simulink model "ssc_hydromech_power_split_cvt_engine_signal_intf"  (R2025a)
settings: Solver=ode23t  StartTime=0.0  StopTime=70  RelTol=1e-3  AbsTol=1e-3
StartFcn:
  | tic
StopFcn:
  | Elapsed_Sim_Time = toc;
  | disp(['Elapsed Sim Time = ' num2str(Elapsed_Sim_Time)]);
undefined symbols (not defined in the file): DiscIntNeverNeededParam, HMPST, K, Lambda, tau, x0
libraries: fl_lib x30, nesl_utility x16, sm_wheel_loader_lib x9, simulink x7, simulink_extras x6, sdl_lib x3
(part 3 of 4)

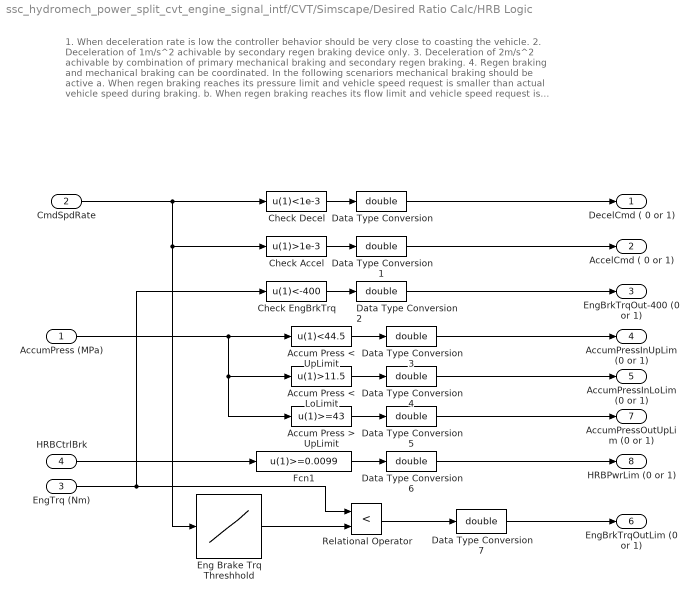
== system ssc_hydromech_power_split_cvt_engine_signal_intf/CVT/Simscape/Desired Ratio Calc/HRB Logic ==
  note: 1. When deceleration rate is low the controller behavior should be very close to coasting the vehicle.
      | 2. Deceleration of 1m/s^2 achivable by secondary regen braking device only.
      | 3. Deceleration of 2m/s^2 achivable by combination of primary mechanical braking and secondary regen braking.
      | 4. Regen braking and mechanical braking can be coordinated. In the following scenariors mechanical braking should be active
      | a. When regen braking reaches its pressure limit and vehicle speed request is smaller than actual vehicle speed during braking.
      | b. When regen braking reaches its flow limit and vehicle speed request is smaller than actual vehicle speed during braking.
      | 5. Energy in the accumulator will be released when accelerating and the accumulator pressure is above minimum working pressure.
      | Energy release rate should not cause engine over speeding.
      | 6. If engine over speed limit is reached disengage master clutch/shut down the engine.
  AccumPress (MPa) : Inport
  CmdSpdRate : Inport  Port=2
  EngTrq (Nm) : Inport  Port=3
  HRBCtrlBrk : Inport  Port=4
  Accum Press < LoLimit : Fcn  Expr=u(1)>11.5
  Accum Press < UpLimit : Fcn  Expr=u(1)<44.5
  Accum Press > UpLimit : Fcn  Expr=u(1)>=43
  Check Accel : Fcn  Expr=u(1)>1e-3
  Check Decel : Fcn  Expr=u(1)<1e-3
  Check EngBrkTrq : Fcn  Expr=u(1)<-400
  Data Type Conversion{,1..7} (8 alike) : DataTypeConversion  OutDataTypeStr=double  SaturateOnIntegerOverflow=off  RndMeth=Floor
  Eng Brake Trq Threshhold : Lookup_n-D  NumberOfTableDimensions=1  BreakpointsForDimension1=[-3 -2 -1 -0.5 0 1]  Table=[-450 -450 -225 -113 0 0]*0.6  InternalRulePriority=Speed  RndMeth=Simplest
  Fcn1 : Fcn  Expr=u(1)>=0.0099
  Relational Operator : RelationalOperator  Operator=<  OutDataTypeStr=boolean  ZeroCross=off  InputSameDT=off
  DecelCmd ( 0 or 1) : Outport
  AccelCmd ( 0 or 1) : Outport  Port=2
  EngBrkTrqOut-400 (0 or 1) : Outport  Port=3
  AccumPressInUpLim (0 or 1) : Outport  Port=4
  AccumPressInLoLim (0 or 1) : Outport  Port=5
  EngBrkTrqOutLim (0 or 1) : Outport  Port=6
  AccumPressOutUpLim (0 or 1) : Outport  Port=7
  HRBPwrLim (0 or 1) : Outport  Port=8
  wires:
  Data Type Conversion7/1 -> EngBrkTrqOutLim (0 or 1)/1
  Data Type Conversion6/1 -> HRBPwrLim (0 or 1)/1
  Data Type Conversion5/1 -> AccumPressOutUpLim (0 or 1)/1
  Data Type Conversion4/1 -> AccumPressInLoLim (0 or 1)/1
  Data Type Conversion3/1 -> AccumPressInUpLim (0 or 1)/1
  Data Type Conversion2/1 -> EngBrkTrqOut-400 (0 or 1)/1
  Data Type Conversion1/1 -> AccelCmd ( 0 or 1)/1
  Check EngBrkTrq/1 -> Data Type Conversion2/1
  Check Accel/1 -> Data Type Conversion1/1
  Accum Press < LoLimit/1 -> Data Type Conversion4/1
  Fcn1/1 -> Data Type Conversion6/1
  HRBCtrlBrk/1 -> Fcn1/1
  Accum Press > UpLimit/1 -> Data Type Conversion5/1
  Relational Operator/1 -> Data Type Conversion7/1
  Accum Press < UpLimit/1 -> Data Type Conversion3/1
  AccumPress (MPa)/1 -> Accum Press < UpLimit/1, Accum Press > UpLimit/1, Accum Press < LoLimit/1
  Eng Brake Trq Threshhold/1 -> Relational Operator/2
  CmdSpdRate/1 -> Check Accel/1, Eng Brake Trq Threshhold/1, Check Decel/1
  EngTrq (Nm)/1 -> Check EngBrkTrq/1, Relational Operator/1
  Data Type Conversion/1 -> DecelCmd ( 0 or 1)/1
  Check Decel/1 -> Data Type Conversion/1

== system ssc_hydromech_power_split_cvt_engine_signal_intf/CVT/Simscape/Desired Ratio Calc/MB Control ==
  Decel Error : Inport
  wTransOutCmd : Inport  Port=2
  Rset : Inport  Port=3
  AccumLimUp : Inport  Port=4
  HRBPowerLim : Inport  Port=5
  Add1 : Sum  Inputs=+++
  Compare To Constant : simulink/Logic and Bit Operations/Compare To Constant  relop=<=  const=0.02  OutDataTypeStr=boolean
  Data Type Conversion : DataTypeConversion  OutDataTypeStr=double  SaturateOnIntegerOverflow=off  RndMeth=Floor
  PI MB No HRB : Subsystem
  PI MB with MRB : Subsystem
  Product3 : Product  Inputs=3
  Product4 : Product
  Out1 : Outport
  wires:
  Decel Error/1 -> Product3/1, Product4/1
  Product3/1 -> PI MB No HRB/1(error)
  Rset/1 -> Product3/2, PI MB No HRB/2(Rset), PI MB with MRB/2(Rset)
  Compare To Constant/1 -> Data Type Conversion/1
  Data Type Conversion/1 -> Add1/1
  PI MB No HRB/1(ctrl) -> Add1/2
  Product4/1 -> PI MB with MRB/1(error)
  Add1/1 -> Out1/1
  PI MB with MRB/1(ctrl) -> Add1/3
  wTransOutCmd/1 -> Compare To Constant/1
  AccumLimUp/1 -> Product3/3
  HRBPowerLim/1 -> Product4/2

== system ssc_hydromech_power_split_cvt_engine_signal_intf/CVT/Simscape/Desired Ratio Calc/Subsystem ==
  u : Inport
  Constant1 : Constant
  Constant2 : Constant  Value=-1
  Constant3 : Constant  Value=0
  Gain : Gain  Gain=-1
  Switch : Switch  Criteria=u2 > Threshold  Threshold=0.001  SaturateOnIntegerOverflow=off  InputSameDT=off
  Switch1 : Switch  Criteria=u2 > Threshold  Threshold=0.001  SaturateOnIntegerOverflow=off  InputSameDT=off
  u_dir : Outport
  wires:
  Constant2/1 -> Switch1/1
  Constant3/1 -> Switch1/3
  Switch1/1 -> Switch/3
  Constant1/1 -> Switch/1
  u/1 -> Gain/1, Switch/2
  Switch/1 -> u_dir/1
  Gain/1 -> Switch1/2

== system ssc_hydromech_power_split_cvt_engine_signal_intf/CVT/Simscape/Port 1 Interface Engine/Interface ==
  across1 : Inport
  across2 : Inport  Port=2
  Continuous : Subsystem  VariantControl=Continuous
  Discrete : Subsystem  VariantControl=Discrete
  through2 : Outport
  through1 : Outport  Port=2

== system ssc_hydromech_power_split_cvt_engine_signal_intf/CVT/Simscape/Port 1 Interface Vehicle/Interface ==
  across1 : Inport
  across2 : Inport  Port=2
  Continuous : Subsystem  VariantControl=Continuous
  Discrete : Subsystem  VariantControl=Discrete
  through2 : Outport
  through1 : Outport  Port=2

== system ssc_hydromech_power_split_cvt_engine_signal_intf/CVT/Other/Desired Ratio Calc/HRB Control/PI HRB Brake ==
  error : Inport
  Rset : Inport  Port=2
  Gain : Gain  Gain=0.02*0.2
  Gain3 : Gain  Gain=0.002+0.0005
  Integrator : Integrator  ExternalReset=falling
  Sum : Sum  Inputs=++|
  ctrl : Outport
  wires:
  Rset/1 -> Integrator/2
  Integrator/1 -> Sum/1
  error/1 -> Gain3/1, Gain/1
  Sum/1 -> ctrl/1
  Gain3/1 -> Integrator/1
  Gain/1 -> Sum/2

== system ssc_hydromech_power_split_cvt_engine_signal_intf/CVT/Other/Desired Ratio Calc/HRB Control/PI HRB Regen ==
  error : Inport
  Rset : Inport  Port=2
  Gain : Gain  Gain=0.01*0.2
  Gain3 : Gain  Gain=0.001
  Integrator : Integrator  ExternalReset=falling
  Sum : Sum  Inputs=++|
  ctrl : Outport
  wires:
  Gain/1 -> Sum/2
  Gain3/1 -> Integrator/1
  Sum/1 -> ctrl/1
  error/1 -> Gain/1, Gain3/1
  Integrator/1 -> Sum/1
  Rset/1 -> Integrator/2

== system ssc_hydromech_power_split_cvt_engine_signal_intf/CVT/Other/Desired Ratio Calc/MB Control/PI MB No HRB ==
  error : Inport
  Rset : Inport  Port=2
  Gain : Gain  Gain=0.01
  Gain3 : Gain  Gain=0.002
  Integrator : Integrator  ExternalReset=falling
  Sum : Sum  Inputs=++|
  ctrl : Outport
  wires:
  Rset/1 -> Integrator/2
  Integrator/1 -> Sum/1
  error/1 -> Gain3/1, Gain/1
  Sum/1 -> ctrl/1
  Gain3/1 -> Integrator/1
  Gain/1 -> Sum/2

== system ssc_hydromech_power_split_cvt_engine_signal_intf/CVT/Other/Desired Ratio Calc/MB Control/PI MB with MRB ==
  error : Inport
  Rset : Inport  Port=2
  Gain : Gain  Gain=0.005
  Gain3 : Gain  Gain=0.002
  Integrator : Integrator  ExternalReset=falling
  Sum : Sum  Inputs=++|
  ctrl : Outport
  wires:
  Gain/1 -> Sum/2
  Gain3/1 -> Integrator/1
  Sum/1 -> ctrl/1
  error/1 -> Gain/1, Gain3/1
  Integrator/1 -> Sum/1
  Rset/1 -> Integrator/2

== system ssc_hydromech_power_split_cvt_engine_signal_intf/CVT/Other/Port 1 Interface Engine/Interface/Continuous ==
  across2 : Inport
  across1 : Inport  Port=2
  -1 : Gain  Gain=-1  SaturateOnIntegerOverflow=on  OutDataTypeStr=Inherit: Same as input  ParamDataTypeStr=Inherit: Same as input
  Integrator : Integrator  InitialCondition=x0
  K : Gain  Gain=K  SaturateOnIntegerOverflow=on  OutDataTypeStr=Inherit: Same as input  ParamDataTypeStr=Inherit: Same as input
  Lambda : Gain  Gain=Lambda  SaturateOnIntegerOverflow=on  OutDataTypeStr=Inherit: Same as input  ParamDataTypeStr=Inherit: Same as input
  Low-pass filter : TransferFcn  Numerator=1  Denominator=[tau 1]
  Prediction : Subsystem  Commented=through  mask(Prediction (discrete->continuous)){h2=h2}
      mask prompts: h2 "physmod:simscape:couplers:SimscapeNetworkCouplersLib:PortUDiscreteSampleTimes_MP"
      mask help: physmod:simscape:couplers:SimscapeNetworkCouplersLib:Predictiondiscretecontinuous_MD
      mask DialogControl h2 Prompt: Port u discrete sample time (s)
  Smoothing : Subsystem  Commented=through  mask(Smoothing (continuous->discrete)){tsSmoothing=tsSmoothing, smoothing0=-through0}
      mask prompts: tsSmoothing "physmod:simscape:couplers:SimscapeNetworkCouplersLib:SmoothingTimeConstants_MP"; smoothing0 "physmod:simscape:couplers:SimscapeNetworkCouplersLib:InitialOutput_MP"
      mask help: physmod:simscape:couplers:SimscapeNetworkCouplersLib:Smoothingcontinuousdiscrete_MD
      mask DialogControl tsSmoothing Prompt: Smoothing time constant (s)
      mask DialogControl smoothing0 Prompt: Initial output
  Sum : Sum  Inputs=+-  InputSameDT=on  SaturateOnIntegerOverflow=on  OutDataTypeStr=Inherit: Same as first input
  Sum2 : Sum  Inputs=|++
  through2 : Outport
  through1 : Outport  Port=2
  wires:
  K/1 -> Sum2/1
  Sum2/1 -> through1/1, -1/1
  across2/1 -> Prediction/1(u)
  Low-pass filter/1 -> Lambda/1
  Integrator/1 -> K/1
  Sum/1 -> Integrator/1, Low-pass filter/1
  across1/1 -> Sum/1
  Lambda/1 -> Sum2/2
  Prediction/1(y) -> Sum/2
  Smoothing/1(y) -> through2/1
  -1/1 -> Smoothing/1(u)

== system ssc_hydromech_power_split_cvt_engine_signal_intf/CVT/Other/Port 1 Interface Engine/Interface/Discrete ==
  across2 : Inport
  across1 : Inport  Port=2
  -1 : Gain  Gain=-1  SaturateOnIntegerOverflow=on  OutDataTypeStr=Inherit: Same as input  ParamDataTypeStr=Inherit: Same as input
  First-order lag : DiscreteTransferFcn  Numerator=h1  Denominator=[tau h1-tau]  SampleTime=h1
  Integrator : DiscreteIntegrator  InitialCondition=x0  SampleTime=h1  ICPrevOutput=DiscIntNeverNeededParam  ICPrevScaledInput=DiscIntNeverNeededParam
  K : Gain  Gain=K  SaturateOnIntegerOverflow=on  OutDataTypeStr=Inherit: Same as input  ParamDataTypeStr=Inherit: Same as input
  Lambda : Gain  Gain=Lambda  SaturateOnIntegerOverflow=on  OutDataTypeStr=Inherit: Same as input  ParamDataTypeStr=Inherit: Same as input
  Prediction : Subsystem  Commented=through  mask(Prediction (slow->fast)){h2=h2, h1=h1}
      mask prompts: h2 "physmod:simscape:couplers:SimscapeNetworkCouplersLib:PortUDiscreteSampleTimes_MP"; h1 "physmod:simscape:couplers:SimscapeNetworkCouplersLib:PortYDiscreteSampleTimes_MP"
      mask help: physmod:simscape:couplers:SimscapeNetworkCouplersLib:Predictionslowfast_MD
      mask DialogControl h2 Prompt: Port u discrete sample time (s)
      mask DialogControl h1 Prompt: Port y discrete sample time (s)
  Smoothing : Subsystem  Commented=through  mask(Smoothing (fast->slow)){nSmooth=nSmooth, h1=h1, smoothing0=-through0}
      mask prompts: nSmooth "physmod:simscape:couplers:SimscapeNetworkCouplersLib:NumberOfSamplesOverWhichToSmooth_MP"; h1 "physmod:simscape:couplers:SimscapeNetworkCouplersLib:PortUDiscreteSampleTimes_MP"; smoothing0 "physmod:simscape:couplers:SimscapeNetworkCouplersLib:InitialOutput_MP"
      mask help: physmod:simscape:couplers:SimscapeNetworkCouplersLib:Smoothingfastslow_MD
      mask DialogControl nSmooth Prompt: Number of samples over which to smooth
      mask DialogControl h1 Prompt: Port u discrete sample time (s)
      mask DialogControl smoothing0 Prompt: Initial output
  Sum : Sum  Inputs=+-  InputSameDT=on  SaturateOnIntegerOverflow=on  OutDataTypeStr=Inherit: Same as first input
  Sum1 : Sum  Inputs=|++
  through2 : Outport
  through1 : Outport  Port=2
  wires:
  First-order lag/1 -> Lambda/1
  Integrator/1 -> K/1
  K/1 -> Sum1/1
  across1/1 -> Sum/1
  Sum/1 -> Integrator/1, First-order lag/1
  across2/1 -> Prediction/1(u)
  Sum1/1 -> through1/1, -1/1
  Lambda/1 -> Sum1/2
  Prediction/1(y) -> Sum/2
  Smoothing/1(y) -> through2/1
  -1/1 -> Smoothing/1(u)

== system ssc_hydromech_power_split_cvt_engine_signal_intf/CVT/Other/Port 1 Interface Vehicle/Interface/Continuous ==
  across2 : Inport
  across1 : Inport  Port=2
  -1 : Gain  Gain=-1  SaturateOnIntegerOverflow=on  OutDataTypeStr=Inherit: Same as input  ParamDataTypeStr=Inherit: Same as input
  Integrator : Integrator  InitialCondition=x0
  K : Gain  Gain=K  SaturateOnIntegerOverflow=on  OutDataTypeStr=Inherit: Same as input  ParamDataTypeStr=Inherit: Same as input
  Lambda : Gain  Gain=Lambda  SaturateOnIntegerOverflow=on  OutDataTypeStr=Inherit: Same as input  ParamDataTypeStr=Inherit: Same as input
  Low-pass filter : TransferFcn  Numerator=1  Denominator=[tau 1]
  Prediction : Subsystem  Commented=through  mask(Prediction (discrete->continuous)){h2=h2}
      mask prompts: h2 "physmod:simscape:couplers:SimscapeNetworkCouplersLib:PortUDiscreteSampleTimes_MP"
      mask help: physmod:simscape:couplers:SimscapeNetworkCouplersLib:Predictiondiscretecontinuous_MD
      mask DialogControl h2 Prompt: Port u discrete sample time (s)
  Smoothing : Subsystem  Commented=through  mask(Smoothing (continuous->discrete)){tsSmoothing=tsSmoothing, smoothing0=-through0}
      mask prompts: tsSmoothing "physmod:simscape:couplers:SimscapeNetworkCouplersLib:SmoothingTimeConstants_MP"; smoothing0 "physmod:simscape:couplers:SimscapeNetworkCouplersLib:InitialOutput_MP"
      mask help: physmod:simscape:couplers:SimscapeNetworkCouplersLib:Smoothingcontinuousdiscrete_MD
      mask DialogControl tsSmoothing Prompt: Smoothing time constant (s)
      mask DialogControl smoothing0 Prompt: Initial output
  Sum : Sum  Inputs=+-  InputSameDT=on  SaturateOnIntegerOverflow=on  OutDataTypeStr=Inherit: Same as first input
  Sum2 : Sum  Inputs=|++
  through2 : Outport
  through1 : Outport  Port=2
  wires:
  K/1 -> Sum2/1
  Sum2/1 -> through1/1, -1/1
  across2/1 -> Prediction/1(u)
  Low-pass filter/1 -> Lambda/1
  Integrator/1 -> K/1
  Sum/1 -> Integrator/1, Low-pass filter/1
  across1/1 -> Sum/1
  Lambda/1 -> Sum2/2
  Prediction/1(y) -> Sum/2
  Smoothing/1(y) -> through2/1
  -1/1 -> Smoothing/1(u)

== system ssc_hydromech_power_split_cvt_engine_signal_intf/CVT/Other/Port 1 Interface Vehicle/Interface/Discrete ==
  across2 : Inport
  across1 : Inport  Port=2
  -1 : Gain  Gain=-1  SaturateOnIntegerOverflow=on  OutDataTypeStr=Inherit: Same as input  ParamDataTypeStr=Inherit: Same as input
  First-order lag : DiscreteTransferFcn  Numerator=h1  Denominator=[tau h1-tau]  SampleTime=h1
  Integrator : DiscreteIntegrator  InitialCondition=x0  SampleTime=h1  ICPrevOutput=DiscIntNeverNeededParam  ICPrevScaledInput=DiscIntNeverNeededParam
  K : Gain  Gain=K  SaturateOnIntegerOverflow=on  OutDataTypeStr=Inherit: Same as input  ParamDataTypeStr=Inherit: Same as input
  Lambda : Gain  Gain=Lambda  SaturateOnIntegerOverflow=on  OutDataTypeStr=Inherit: Same as input  ParamDataTypeStr=Inherit: Same as input
  Prediction : Subsystem  Commented=through  mask(Prediction (slow->fast)){h2=h2, h1=h1}
      mask prompts: h2 "physmod:simscape:couplers:SimscapeNetworkCouplersLib:PortUDiscreteSampleTimes_MP"; h1 "physmod:simscape:couplers:SimscapeNetworkCouplersLib:PortYDiscreteSampleTimes_MP"
      mask help: physmod:simscape:couplers:SimscapeNetworkCouplersLib:Predictionslowfast_MD
      mask DialogControl h2 Prompt: Port u discrete sample time (s)
      mask DialogControl h1 Prompt: Port y discrete sample time (s)
  Smoothing : Subsystem  Commented=through  mask(Smoothing (fast->slow)){nSmooth=nSmooth, h1=h1, smoothing0=-through0}
      mask prompts: nSmooth "physmod:simscape:couplers:SimscapeNetworkCouplersLib:NumberOfSamplesOverWhichToSmooth_MP"; h1 "physmod:simscape:couplers:SimscapeNetworkCouplersLib:PortUDiscreteSampleTimes_MP"; smoothing0 "physmod:simscape:couplers:SimscapeNetworkCouplersLib:InitialOutput_MP"
      mask help: physmod:simscape:couplers:SimscapeNetworkCouplersLib:Smoothingfastslow_MD
      mask DialogControl nSmooth Prompt: Number of samples over which to smooth
      mask DialogControl h1 Prompt: Port u discrete sample time (s)
      mask DialogControl smoothing0 Prompt: Initial output
  Sum : Sum  Inputs=+-  InputSameDT=on  SaturateOnIntegerOverflow=on  OutDataTypeStr=Inherit: Same as first input
  Sum1 : Sum  Inputs=|++
  through2 : Outport
  through1 : Outport  Port=2
  wires:
  First-order lag/1 -> Lambda/1
  Integrator/1 -> K/1
  K/1 -> Sum1/1
  across1/1 -> Sum/1
  Sum/1 -> Integrator/1, First-order lag/1
  across2/1 -> Prediction/1(u)
  Sum1/1 -> through1/1, -1/1
  Lambda/1 -> Sum1/2
  Prediction/1(y) -> Sum/2
  Smoothing/1(y) -> through2/1
  -1/1 -> Smoothing/1(u)

== system ssc_hydromech_power_split_cvt_engine_signal_intf/CVT/Simscape/Desired Ratio Calc/HRB Control/PI HRB Brake ==
  error : Inport
  Rset : Inport  Port=2
  Gain : Gain  Gain=0.02*0.2
  Gain3 : Gain  Gain=0.002+0.0005
  Integrator : Integrator  ExternalReset=falling
  Sum : Sum  Inputs=++|
  ctrl : Outport
  wires:
  Gain/1 -> Sum/2
  Gain3/1 -> Integrator/1
  Sum/1 -> ctrl/1
  error/1 -> Gain/1, Gain3/1
  Integrator/1 -> Sum/1
  Rset/1 -> Integrator/2

== system ssc_hydromech_power_split_cvt_engine_signal_intf/CVT/Simscape/Desired Ratio Calc/HRB Control/PI HRB Regen ==
  error : Inport
  Rset : Inport  Port=2
  Gain : Gain  Gain=0.01*0.2
  Gain3 : Gain  Gain=0.001
  Integrator : Integrator  ExternalReset=falling
  Sum : Sum  Inputs=++|
  ctrl : Outport
  wires:
  Rset/1 -> Integrator/2
  Integrator/1 -> Sum/1
  error/1 -> Gain3/1, Gain/1
  Sum/1 -> ctrl/1
  Gain3/1 -> Integrator/1
  Gain/1 -> Sum/2

== system ssc_hydromech_power_split_cvt_engine_signal_intf/CVT/Simscape/Desired Ratio Calc/MB Control/PI MB No HRB ==
  error : Inport
  Rset : Inport  Port=2
  Gain : Gain  Gain=0.01
  Gain3 : Gain  Gain=0.002
  Integrator : Integrator  ExternalReset=falling
  Sum : Sum  Inputs=++|
  ctrl : Outport
  wires:
  Gain/1 -> Sum/2
  Gain3/1 -> Integrator/1
  Sum/1 -> ctrl/1
  error/1 -> Gain/1, Gain3/1
  Integrator/1 -> Sum/1
  Rset/1 -> Integrator/2

== system ssc_hydromech_power_split_cvt_engine_signal_intf/CVT/Simscape/Desired Ratio Calc/MB Control/PI MB with MRB ==
  error : Inport
  Rset : Inport  Port=2
  Gain : Gain  Gain=0.005
  Gain3 : Gain  Gain=0.002
  Integrator : Integrator  ExternalReset=falling
  Sum : Sum  Inputs=++|
  ctrl : Outport
  wires:
  Rset/1 -> Integrator/2
  Integrator/1 -> Sum/1
  error/1 -> Gain3/1, Gain/1
  Sum/1 -> ctrl/1
  Gain3/1 -> Integrator/1
  Gain/1 -> Sum/2

== system ssc_hydromech_power_split_cvt_engine_signal_intf/CVT/Simscape/Port 1 Interface Engine/Interface/Continuous ==
  across2 : Inport
  across1 : Inport  Port=2
  -1 : Gain  Gain=-1  SaturateOnIntegerOverflow=on  OutDataTypeStr=Inherit: Same as input  ParamDataTypeStr=Inherit: Same as input
  Integrator : Integrator  InitialCondition=x0
  K : Gain  Gain=K  SaturateOnIntegerOverflow=on  OutDataTypeStr=Inherit: Same as input  ParamDataTypeStr=Inherit: Same as input
  Lambda : Gain  Gain=Lambda  SaturateOnIntegerOverflow=on  OutDataTypeStr=Inherit: Same as input  ParamDataTypeStr=Inherit: Same as input
  Low-pass filter : TransferFcn  Numerator=1  Denominator=[tau 1]
  Prediction : Subsystem  Commented=through  mask(Prediction (discrete->continuous)){h2=h2}
      mask prompts: h2 "physmod:simscape:couplers:SimscapeNetworkCouplersLib:PortUDiscreteSampleTimes_MP"
      mask help: physmod:simscape:couplers:SimscapeNetworkCouplersLib:Predictiondiscretecontinuous_MD
      mask DialogControl h2 Prompt: Port u discrete sample time (s)
  Smoothing : Subsystem  Commented=through  mask(Smoothing (continuous->discrete)){tsSmoothing=tsSmoothing, smoothing0=-through0}
      mask prompts: tsSmoothing "physmod:simscape:couplers:SimscapeNetworkCouplersLib:SmoothingTimeConstants_MP"; smoothing0 "physmod:simscape:couplers:SimscapeNetworkCouplersLib:InitialOutput_MP"
      mask help: physmod:simscape:couplers:SimscapeNetworkCouplersLib:Smoothingcontinuousdiscrete_MD
      mask DialogControl tsSmoothing Prompt: Smoothing time constant (s)
      mask DialogControl smoothing0 Prompt: Initial output
  Sum : Sum  Inputs=+-  InputSameDT=on  SaturateOnIntegerOverflow=on  OutDataTypeStr=Inherit: Same as first input
  Sum2 : Sum  Inputs=|++
  through2 : Outport
  through1 : Outport  Port=2
  wires:
  -1/1 -> Smoothing/1(u)
  Smoothing/1(y) -> through2/1
  Prediction/1(y) -> Sum/2
  Lambda/1 -> Sum2/2
  across1/1 -> Sum/1
  Sum/1 -> Low-pass filter/1, Integrator/1
  Integrator/1 -> K/1
  Low-pass filter/1 -> Lambda/1
  across2/1 -> Prediction/1(u)
  Sum2/1 -> -1/1, through1/1
  K/1 -> Sum2/1

== system ssc_hydromech_power_split_cvt_engine_signal_intf/CVT/Simscape/Port 1 Interface Engine/Interface/Discrete ==
  across2 : Inport
  across1 : Inport  Port=2
  -1 : Gain  Gain=-1  SaturateOnIntegerOverflow=on  OutDataTypeStr=Inherit: Same as input  ParamDataTypeStr=Inherit: Same as input
  First-order lag : DiscreteTransferFcn  Numerator=h1  Denominator=[tau h1-tau]  SampleTime=h1
  Integrator : DiscreteIntegrator  InitialCondition=x0  SampleTime=h1  ICPrevOutput=DiscIntNeverNeededParam  ICPrevScaledInput=DiscIntNeverNeededParam
  K : Gain  Gain=K  SaturateOnIntegerOverflow=on  OutDataTypeStr=Inherit: Same as input  ParamDataTypeStr=Inherit: Same as input
  Lambda : Gain  Gain=Lambda  SaturateOnIntegerOverflow=on  OutDataTypeStr=Inherit: Same as input  ParamDataTypeStr=Inherit: Same as input
  Prediction : Subsystem  Commented=through  mask(Prediction (slow->fast)){h2=h2, h1=h1}
      mask prompts: h2 "physmod:simscape:couplers:SimscapeNetworkCouplersLib:PortUDiscreteSampleTimes_MP"; h1 "physmod:simscape:couplers:SimscapeNetworkCouplersLib:PortYDiscreteSampleTimes_MP"
      mask help: physmod:simscape:couplers:SimscapeNetworkCouplersLib:Predictionslowfast_MD
      mask DialogControl h2 Prompt: Port u discrete sample time (s)
      mask DialogControl h1 Prompt: Port y discrete sample time (s)
  Smoothing : Subsystem  Commented=through  mask(Smoothing (fast->slow)){nSmooth=nSmooth, h1=h1, smoothing0=-through0}
      mask prompts: nSmooth "physmod:simscape:couplers:SimscapeNetworkCouplersLib:NumberOfSamplesOverWhichToSmooth_MP"; h1 "physmod:simscape:couplers:SimscapeNetworkCouplersLib:PortUDiscreteSampleTimes_MP"; smoothing0 "physmod:simscape:couplers:SimscapeNetworkCouplersLib:InitialOutput_MP"
      mask help: physmod:simscape:couplers:SimscapeNetworkCouplersLib:Smoothingfastslow_MD
      mask DialogControl nSmooth Prompt: Number of samples over which to smooth
      mask DialogControl h1 Prompt: Port u discrete sample time (s)
      mask DialogControl smoothing0 Prompt: Initial output
  Sum : Sum  Inputs=+-  InputSameDT=on  SaturateOnIntegerOverflow=on  OutDataTypeStr=Inherit: Same as first input
  Sum1 : Sum  Inputs=|++
  through2 : Outport
  through1 : Outport  Port=2
  wires:
  -1/1 -> Smoothing/1(u)
  Smoothing/1(y) -> through2/1
  Prediction/1(y) -> Sum/2
  Lambda/1 -> Sum1/2
  Sum1/1 -> -1/1, through1/1
  across2/1 -> Prediction/1(u)
  Sum/1 -> First-order lag/1, Integrator/1
  across1/1 -> Sum/1
  K/1 -> Sum1/1
  Integrator/1 -> K/1
  First-order lag/1 -> Lambda/1

== system ssc_hydromech_power_split_cvt_engine_signal_intf/CVT/Simscape/Port 1 Interface Vehicle/Interface/Continuous ==
  across2 : Inport
  across1 : Inport  Port=2
  -1 : Gain  Gain=-1  SaturateOnIntegerOverflow=on  OutDataTypeStr=Inherit: Same as input  ParamDataTypeStr=Inherit: Same as input
  Integrator : Integrator  InitialCondition=x0
  K : Gain  Gain=K  SaturateOnIntegerOverflow=on  OutDataTypeStr=Inherit: Same as input  ParamDataTypeStr=Inherit: Same as input
  Lambda : Gain  Gain=Lambda  SaturateOnIntegerOverflow=on  OutDataTypeStr=Inherit: Same as input  ParamDataTypeStr=Inherit: Same as input
  Low-pass filter : TransferFcn  Numerator=1  Denominator=[tau 1]
  Prediction : Subsystem  Commented=through  mask(Prediction (discrete->continuous)){h2=h2}
      mask prompts: h2 "physmod:simscape:couplers:SimscapeNetworkCouplersLib:PortUDiscreteSampleTimes_MP"
      mask help: physmod:simscape:couplers:SimscapeNetworkCouplersLib:Predictiondiscretecontinuous_MD
      mask DialogControl h2 Prompt: Port u discrete sample time (s)
  Smoothing : Subsystem  Commented=through  mask(Smoothing (continuous->discrete)){tsSmoothing=tsSmoothing, smoothing0=-through0}
      mask prompts: tsSmoothing "physmod:simscape:couplers:SimscapeNetworkCouplersLib:SmoothingTimeConstants_MP"; smoothing0 "physmod:simscape:couplers:SimscapeNetworkCouplersLib:InitialOutput_MP"
      mask help: physmod:simscape:couplers:SimscapeNetworkCouplersLib:Smoothingcontinuousdiscrete_MD
      mask DialogControl tsSmoothing Prompt: Smoothing time constant (s)
      mask DialogControl smoothing0 Prompt: Initial output
  Sum : Sum  Inputs=+-  InputSameDT=on  SaturateOnIntegerOverflow=on  OutDataTypeStr=Inherit: Same as first input
  Sum2 : Sum  Inputs=|++
  through2 : Outport
  through1 : Outport  Port=2
  wires:
  -1/1 -> Smoothing/1(u)
  Smoothing/1(y) -> through2/1
  Prediction/1(y) -> Sum/2
  Lambda/1 -> Sum2/2
  across1/1 -> Sum/1
  Sum/1 -> Low-pass filter/1, Integrator/1
  Integrator/1 -> K/1
  Low-pass filter/1 -> Lambda/1
  across2/1 -> Prediction/1(u)
  Sum2/1 -> -1/1, through1/1
  K/1 -> Sum2/1

== system ssc_hydromech_power_split_cvt_engine_signal_intf/CVT/Simscape/Port 1 Interface Vehicle/Interface/Discrete ==
  across2 : Inport
  across1 : Inport  Port=2
  -1 : Gain  Gain=-1  SaturateOnIntegerOverflow=on  OutDataTypeStr=Inherit: Same as input  ParamDataTypeStr=Inherit: Same as input
  First-order lag : DiscreteTransferFcn  Numerator=h1  Denominator=[tau h1-tau]  SampleTime=h1
  Integrator : DiscreteIntegrator  InitialCondition=x0  SampleTime=h1  ICPrevOutput=DiscIntNeverNeededParam  ICPrevScaledInput=DiscIntNeverNeededParam
  K : Gain  Gain=K  SaturateOnIntegerOverflow=on  OutDataTypeStr=Inherit: Same as input  ParamDataTypeStr=Inherit: Same as input
  Lambda : Gain  Gain=Lambda  SaturateOnIntegerOverflow=on  OutDataTypeStr=Inherit: Same as input  ParamDataTypeStr=Inherit: Same as input
  Prediction : Subsystem  Commented=through  mask(Prediction (slow->fast)){h2=h2, h1=h1}
      mask prompts: h2 "physmod:simscape:couplers:SimscapeNetworkCouplersLib:PortUDiscreteSampleTimes_MP"; h1 "physmod:simscape:couplers:SimscapeNetworkCouplersLib:PortYDiscreteSampleTimes_MP"
      mask help: physmod:simscape:couplers:SimscapeNetworkCouplersLib:Predictionslowfast_MD
      mask DialogControl h2 Prompt: Port u discrete sample time (s)
      mask DialogControl h1 Prompt: Port y discrete sample time (s)
  Smoothing : Subsystem  Commented=through  mask(Smoothing (fast->slow)){nSmooth=nSmooth, h1=h1, smoothing0=-through0}
      mask prompts: nSmooth "physmod:simscape:couplers:SimscapeNetworkCouplersLib:NumberOfSamplesOverWhichToSmooth_MP"; h1 "physmod:simscape:couplers:SimscapeNetworkCouplersLib:PortUDiscreteSampleTimes_MP"; smoothing0 "physmod:simscape:couplers:SimscapeNetworkCouplersLib:InitialOutput_MP"
      mask help: physmod:simscape:couplers:SimscapeNetworkCouplersLib:Smoothingfastslow_MD
      mask DialogControl nSmooth Prompt: Number of samples over which to smooth
      mask DialogControl h1 Prompt: Port u discrete sample time (s)
      mask DialogControl smoothing0 Prompt: Initial output
  Sum : Sum  Inputs=+-  InputSameDT=on  SaturateOnIntegerOverflow=on  OutDataTypeStr=Inherit: Same as first input
  Sum1 : Sum  Inputs=|++
  through2 : Outport
  through1 : Outport  Port=2
  wires:
  -1/1 -> Smoothing/1(u)
  Smoothing/1(y) -> through2/1
  Prediction/1(y) -> Sum/2
  Lambda/1 -> Sum1/2
  Sum1/1 -> -1/1, through1/1
  across2/1 -> Prediction/1(u)
  Sum/1 -> First-order lag/1, Integrator/1
  across1/1 -> Sum/1
  K/1 -> Sum1/1
  Integrator/1 -> K/1
  First-order lag/1 -> Lambda/1

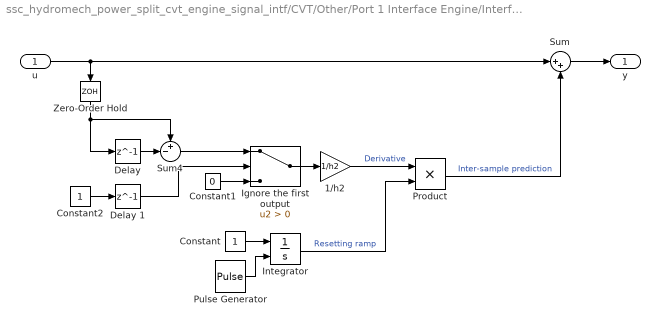
== system ssc_hydromech_power_split_cvt_engine_signal_intf/CVT/Other/Port 1 Interface Engine/Interface/Continuous/Prediction ==
  u : Inport
  1/h2 : Gain  Gain=1/h2
  Constant : Constant  SampleTime=h2
  Constant1 : Constant  Value=0  SampleTime=h2
  Constant2 : Constant  SampleTime=h2
  "Delay " : Delay  DelayLength=1  SampleTime=h2
  Delay 1 : Delay  DelayLength=1  SampleTime=h2
  Ignore the first output : Switch  Criteria=u2 > Threshold  SaturateOnIntegerOverflow=off  InputSameDT=off
  Integrator : Integrator  ExternalReset=either  LimitOutput=on  UpperSaturationLimit=1  LowerSaturationLimit=0
  Product : Product
  Pulse Generator : DiscretePulseGenerator  SampleTime=h2
  Sum : Sum  Inputs=|++
  Sum4 : Sum  Inputs=+-|
  Zero-Order Hold : ZeroOrderHold  SampleTime=h2
  y : Outport
  wires:
  Product/1 -> Sum/2  "Inter-sample prediction"
  Zero-Order Hold/1 -> Sum4/1, "Delay "/1
  u/1 -> Sum/1, Zero-Order Hold/1
  "Delay "/1 -> Sum4/2
  1/h2/1 -> Product/1  "Derivative"
  Sum/1 -> y/1
  Integrator/1 -> Product/2  "Resetting ramp"
  Constant/1 -> Integrator/1
  Pulse Generator/1 -> Integrator/2
  Ignore the first output/1 -> 1/h2/1
  Sum4/1 -> Ignore the first output/1
  Constant1/1 -> Ignore the first output/3
  Delay 1/1 -> Ignore the first output/2
  Constant2/1 -> Delay 1/1

== system ssc_hydromech_power_split_cvt_engine_signal_intf/CVT/Other/Port 1 Interface Engine/Interface/Continuous/Smoothing ==
  u : Inport
  Gain : Gain  Gain=1/tsSmoothing
  Integrator : Integrator  InitialCondition=smoothing0
  Sum : Sum  Inputs=|+-
  y : Outport
  wires:
  u/1 -> Sum/1
  Integrator/1 -> Sum/2, y/1
  Gain/1 -> Integrator/1
  Sum/1 -> Gain/1

== system ssc_hydromech_power_split_cvt_engine_signal_intf/CVT/Other/Port 1 Interface Engine/Interface/Discrete/Prediction ==
  u : Inport
  Abs : Abs  SaturateOnIntegerOverflow=off
  Constant : Constant  Value=0  SampleTime=h1
  Constant2 : Constant  Value=h1  SampleTime=h1
  "Delay " : Delay  DelayLength=1  SampleTime=h1
  Product : Product
  Resettable Delay : Delay  DelayLength=1  InitialConditionSource=Input port  ExternalReset=Rising  SampleTime=h1
      settings: InputPortMap=u0,r5,p4
  Sum : Sum  Inputs=|++
  Sum1 : Sum  Inputs=|++
  Sum2 : Sum  Inputs=+
  Sum4 : Sum  Inputs=+-|
  Update derivative estimate : Subsystem  TreatAsAtomicUnit=on
  y : Outport
  wires:
  Abs/1 -> Sum2/1
  Sum2/1 -> Resettable Delay/2, Update derivative estimate/Trigger  "Trigger when input changes"
  Sum1/1 -> Resettable Delay/1
  Sum/1 -> y/1
  "Delay "/1 -> Sum4/2
  Product/1 -> Sum/2
  Update derivative estimate/1(Out1) -> Product/1
  u/1 -> Update derivative estimate/1(u), "Delay "/1, Sum/1, Sum4/1
  Sum4/1 -> Abs/1
  Resettable Delay/1 -> Product/2, Sum1/2
  Constant2/1 -> Sum1/1
  Constant/1 -> Resettable Delay/3

== system ssc_hydromech_power_split_cvt_engine_signal_intf/CVT/Other/Port 1 Interface Engine/Interface/Discrete/Smoothing ==
  u : Inport
  Gain : Gain  Gain=1/nSmooth
  Sum of Elements : Sum  Inputs=+
  Tapped Delay : simulink/Discrete/Tapped Delay  vinit=smoothing0  samptime=h1  NumDelays=nSmooth  DelayOrder=Oldest  includeCurrent=off
  y : Outport
  wires:
  Gain/1 -> y/1
  Sum of Elements/1 -> Gain/1
  Tapped Delay/1 -> Sum of Elements/1
  u/1 -> Tapped Delay/1

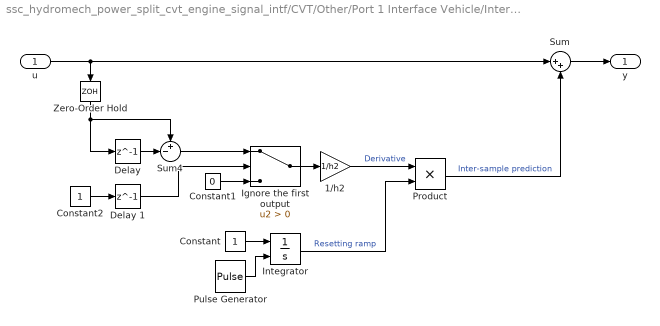
== system ssc_hydromech_power_split_cvt_engine_signal_intf/CVT/Other/Port 1 Interface Vehicle/Interface/Continuous/Prediction ==
  u : Inport
  1/h2 : Gain  Gain=1/h2
  Constant : Constant  SampleTime=h2
  Constant1 : Constant  Value=0  SampleTime=h2
  Constant2 : Constant  SampleTime=h2
  "Delay " : Delay  DelayLength=1  SampleTime=h2
  Delay 1 : Delay  DelayLength=1  SampleTime=h2
  Ignore the first output : Switch  Criteria=u2 > Threshold  SaturateOnIntegerOverflow=off  InputSameDT=off
  Integrator : Integrator  ExternalReset=either  LimitOutput=on  UpperSaturationLimit=1  LowerSaturationLimit=0
  Product : Product
  Pulse Generator : DiscretePulseGenerator  SampleTime=h2
  Sum : Sum  Inputs=|++
  Sum4 : Sum  Inputs=+-|
  Zero-Order Hold : ZeroOrderHold  SampleTime=h2
  y : Outport
  wires:
  Product/1 -> Sum/2  "Inter-sample prediction"
  Zero-Order Hold/1 -> Sum4/1, "Delay "/1
  u/1 -> Sum/1, Zero-Order Hold/1
  "Delay "/1 -> Sum4/2
  1/h2/1 -> Product/1  "Derivative"
  Sum/1 -> y/1
  Integrator/1 -> Product/2  "Resetting ramp"
  Constant/1 -> Integrator/1
  Pulse Generator/1 -> Integrator/2
  Ignore the first output/1 -> 1/h2/1
  Sum4/1 -> Ignore the first output/1
  Constant1/1 -> Ignore the first output/3
  Delay 1/1 -> Ignore the first output/2
  Constant2/1 -> Delay 1/1

== system ssc_hydromech_power_split_cvt_engine_signal_intf/CVT/Other/Port 1 Interface Vehicle/Interface/Continuous/Smoothing ==
  u : Inport
  Gain : Gain  Gain=1/tsSmoothing
  Integrator : Integrator  InitialCondition=smoothing0
  Sum : Sum  Inputs=|+-
  y : Outport
  wires:
  u/1 -> Sum/1
  Integrator/1 -> Sum/2, y/1
  Gain/1 -> Integrator/1
  Sum/1 -> Gain/1

== system ssc_hydromech_power_split_cvt_engine_signal_intf/CVT/Other/Port 1 Interface Vehicle/Interface/Discrete/Prediction ==
  u : Inport
  Abs : Abs  SaturateOnIntegerOverflow=off
  Constant : Constant  Value=0  SampleTime=h1
  Constant2 : Constant  Value=h1  SampleTime=h1
  "Delay " : Delay  DelayLength=1  SampleTime=h1
  Product : Product
  Resettable Delay : Delay  DelayLength=1  InitialConditionSource=Input port  ExternalReset=Rising  SampleTime=h1
      settings: InputPortMap=u0,r5,p4
  Sum : Sum  Inputs=|++
  Sum1 : Sum  Inputs=|++
  Sum2 : Sum  Inputs=+
  Sum4 : Sum  Inputs=+-|
  Update derivative estimate : Subsystem  TreatAsAtomicUnit=on
  y : Outport
  wires:
  Abs/1 -> Sum2/1
  Sum2/1 -> Resettable Delay/2, Update derivative estimate/Trigger  "Trigger when input changes"
  Sum1/1 -> Resettable Delay/1
  Sum/1 -> y/1
  "Delay "/1 -> Sum4/2
  Product/1 -> Sum/2
  Update derivative estimate/1(Out1) -> Product/1
  u/1 -> Update derivative estimate/1(u), "Delay "/1, Sum/1, Sum4/1
  Sum4/1 -> Abs/1
  Resettable Delay/1 -> Product/2, Sum1/2
  Constant2/1 -> Sum1/1
  Constant/1 -> Resettable Delay/3

== system ssc_hydromech_power_split_cvt_engine_signal_intf/CVT/Other/Port 1 Interface Vehicle/Interface/Discrete/Smoothing ==
  u : Inport
  Gain : Gain  Gain=1/nSmooth
  Sum of Elements : Sum  Inputs=+
  Tapped Delay : simulink/Discrete/Tapped Delay  vinit=smoothing0  samptime=h1  NumDelays=nSmooth  DelayOrder=Oldest  includeCurrent=off
  y : Outport
  wires:
  Gain/1 -> y/1
  Sum of Elements/1 -> Gain/1
  Tapped Delay/1 -> Sum of Elements/1
  u/1 -> Tapped Delay/1

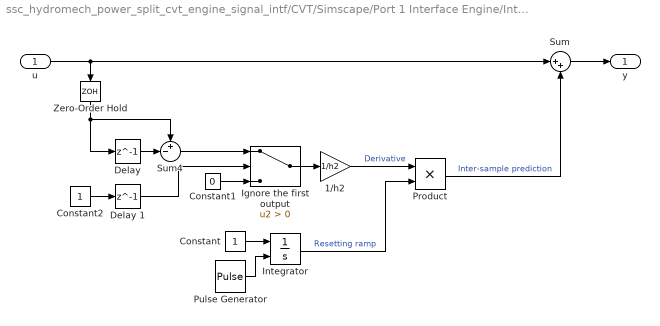
== system ssc_hydromech_power_split_cvt_engine_signal_intf/CVT/Simscape/Port 1 Interface Engine/Interface/Continuous/Prediction ==
  u : Inport
  1/h2 : Gain  Gain=1/h2
  Constant : Constant  SampleTime=h2
  Constant1 : Constant  Value=0  SampleTime=h2
  Constant2 : Constant  SampleTime=h2
  "Delay " : Delay  DelayLength=1  SampleTime=h2
  Delay 1 : Delay  DelayLength=1  SampleTime=h2
  Ignore the first output : Switch  Criteria=u2 > Threshold  SaturateOnIntegerOverflow=off  InputSameDT=off
  Integrator : Integrator  ExternalReset=either  LimitOutput=on  UpperSaturationLimit=1  LowerSaturationLimit=0
  Product : Product
  Pulse Generator : DiscretePulseGenerator  SampleTime=h2
  Sum : Sum  Inputs=|++
  Sum4 : Sum  Inputs=+-|
  Zero-Order Hold : ZeroOrderHold  SampleTime=h2
  y : Outport
  wires:
  Constant2/1 -> Delay 1/1
  Delay 1/1 -> Ignore the first output/2
  Constant1/1 -> Ignore the first output/3
  Sum4/1 -> Ignore the first output/1
  Ignore the first output/1 -> 1/h2/1
  Pulse Generator/1 -> Integrator/2
  Constant/1 -> Integrator/1
  Integrator/1 -> Product/2  "Resetting ramp"
  Sum/1 -> y/1
  1/h2/1 -> Product/1  "Derivative"
  "Delay "/1 -> Sum4/2
  u/1 -> Zero-Order Hold/1, Sum/1
  Zero-Order Hold/1 -> "Delay "/1, Sum4/1
  Product/1 -> Sum/2  "Inter-sample prediction"

== system ssc_hydromech_power_split_cvt_engine_signal_intf/CVT/Simscape/Port 1 Interface Engine/Interface/Continuous/Smoothing ==
  u : Inport
  Gain : Gain  Gain=1/tsSmoothing
  Integrator : Integrator  InitialCondition=smoothing0
  Sum : Sum  Inputs=|+-
  y : Outport
  wires:
  Sum/1 -> Gain/1
  Gain/1 -> Integrator/1
  Integrator/1 -> y/1, Sum/2
  u/1 -> Sum/1

== system ssc_hydromech_power_split_cvt_engine_signal_intf/CVT/Simscape/Port 1 Interface Engine/Interface/Discrete/Prediction ==
  u : Inport
  Abs : Abs  SaturateOnIntegerOverflow=off
  Constant : Constant  Value=0  SampleTime=h1
  Constant2 : Constant  Value=h1  SampleTime=h1
  "Delay " : Delay  DelayLength=1  SampleTime=h1
  Product : Product
  Resettable Delay : Delay  DelayLength=1  InitialConditionSource=Input port  ExternalReset=Rising  SampleTime=h1
      settings: InputPortMap=u0,r5,p4
  Sum : Sum  Inputs=|++
  Sum1 : Sum  Inputs=|++
  Sum2 : Sum  Inputs=+
  Sum4 : Sum  Inputs=+-|
  Update derivative estimate : Subsystem  TreatAsAtomicUnit=on
  y : Outport
  wires:
  Constant/1 -> Resettable Delay/3
  Constant2/1 -> Sum1/1
  Resettable Delay/1 -> Sum1/2, Product/2
  Sum4/1 -> Abs/1
  u/1 -> Sum4/1, Sum/1, "Delay "/1, Update derivative estimate/1(u)
  Update derivative estimate/1(Out1) -> Product/1
  Product/1 -> Sum/2
  "Delay "/1 -> Sum4/2
  Sum/1 -> y/1
  Sum1/1 -> Resettable Delay/1
  Sum2/1 -> Update derivative estimate/Trigger, Resettable Delay/2  "Trigger when input changes"
  Abs/1 -> Sum2/1

== system ssc_hydromech_power_split_cvt_engine_signal_intf/CVT/Simscape/Port 1 Interface Engine/Interface/Discrete/Smoothing ==
  u : Inport
  Gain : Gain  Gain=1/nSmooth
  Sum of Elements : Sum  Inputs=+
  Tapped Delay : simulink/Discrete/Tapped Delay  vinit=smoothing0  samptime=h1  NumDelays=nSmooth  DelayOrder=Oldest  includeCurrent=off
  y : Outport
  wires:
  u/1 -> Tapped Delay/1
  Tapped Delay/1 -> Sum of Elements/1
  Sum of Elements/1 -> Gain/1
  Gain/1 -> y/1

== system ssc_hydromech_power_split_cvt_engine_signal_intf/CVT/Simscape/Port 1 Interface Vehicle/Interface/Continuous/Prediction ==
  u : Inport
  1/h2 : Gain  Gain=1/h2
  Constant : Constant  SampleTime=h2
  Constant1 : Constant  Value=0  SampleTime=h2
  Constant2 : Constant  SampleTime=h2
  "Delay " : Delay  DelayLength=1  SampleTime=h2
  Delay 1 : Delay  DelayLength=1  SampleTime=h2
  Ignore the first output : Switch  Criteria=u2 > Threshold  SaturateOnIntegerOverflow=off  InputSameDT=off
  Integrator : Integrator  ExternalReset=either  LimitOutput=on  UpperSaturationLimit=1  LowerSaturationLimit=0
  Product : Product
  Pulse Generator : DiscretePulseGenerator  SampleTime=h2
  Sum : Sum  Inputs=|++
  Sum4 : Sum  Inputs=+-|
  Zero-Order Hold : ZeroOrderHold  SampleTime=h2
  y : Outport
  wires:
  Constant2/1 -> Delay 1/1
  Delay 1/1 -> Ignore the first output/2
  Constant1/1 -> Ignore the first output/3
  Sum4/1 -> Ignore the first output/1
  Ignore the first output/1 -> 1/h2/1
  Pulse Generator/1 -> Integrator/2
  Constant/1 -> Integrator/1
  Integrator/1 -> Product/2  "Resetting ramp"
  Sum/1 -> y/1
  1/h2/1 -> Product/1  "Derivative"
  "Delay "/1 -> Sum4/2
  u/1 -> Zero-Order Hold/1, Sum/1
  Zero-Order Hold/1 -> "Delay "/1, Sum4/1
  Product/1 -> Sum/2  "Inter-sample prediction"

== system ssc_hydromech_power_split_cvt_engine_signal_intf/CVT/Simscape/Port 1 Interface Vehicle/Interface/Continuous/Smoothing ==
  u : Inport
  Gain : Gain  Gain=1/tsSmoothing
  Integrator : Integrator  InitialCondition=smoothing0
  Sum : Sum  Inputs=|+-
  y : Outport
  wires:
  Sum/1 -> Gain/1
  Gain/1 -> Integrator/1
  Integrator/1 -> y/1, Sum/2
  u/1 -> Sum/1

== system ssc_hydromech_power_split_cvt_engine_signal_intf/CVT/Simscape/Port 1 Interface Vehicle/Interface/Discrete/Prediction ==
  u : Inport
  Abs : Abs  SaturateOnIntegerOverflow=off
  Constant : Constant  Value=0  SampleTime=h1
  Constant2 : Constant  Value=h1  SampleTime=h1
  "Delay " : Delay  DelayLength=1  SampleTime=h1
  Product : Product
  Resettable Delay : Delay  DelayLength=1  InitialConditionSource=Input port  ExternalReset=Rising  SampleTime=h1
      settings: InputPortMap=u0,r5,p4
  Sum : Sum  Inputs=|++
  Sum1 : Sum  Inputs=|++
  Sum2 : Sum  Inputs=+
  Sum4 : Sum  Inputs=+-|
  Update derivative estimate : Subsystem  TreatAsAtomicUnit=on
  y : Outport
  wires:
  Constant/1 -> Resettable Delay/3
  Constant2/1 -> Sum1/1
  Resettable Delay/1 -> Sum1/2, Product/2
  Sum4/1 -> Abs/1
  u/1 -> Sum4/1, Sum/1, "Delay "/1, Update derivative estimate/1(u)
  Update derivative estimate/1(Out1) -> Product/1
  Product/1 -> Sum/2
  "Delay "/1 -> Sum4/2
  Sum/1 -> y/1
  Sum1/1 -> Resettable Delay/1
  Sum2/1 -> Update derivative estimate/Trigger, Resettable Delay/2  "Trigger when input changes"
  Abs/1 -> Sum2/1

== system ssc_hydromech_power_split_cvt_engine_signal_intf/CVT/Simscape/Port 1 Interface Vehicle/Interface/Discrete/Smoothing ==
  u : Inport
  Gain : Gain  Gain=1/nSmooth
  Sum of Elements : Sum  Inputs=+
  Tapped Delay : simulink/Discrete/Tapped Delay  vinit=smoothing0  samptime=h1  NumDelays=nSmooth  DelayOrder=Oldest  includeCurrent=off
  y : Outport
  wires:
  u/1 -> Tapped Delay/1
  Tapped Delay/1 -> Sum of Elements/1
  Sum of Elements/1 -> Gain/1
  Gain/1 -> y/1

== system ssc_hydromech_power_split_cvt_engine_signal_intf/CVT/Other/Port 1 Interface Engine/Interface/Discrete/Prediction/Update derivative estimate ==
  u : Inport
  Trigger : TriggerPort  VariantControl=(inherit)
  1/h2 : Gain  Gain=1/h2
  Constant : Constant  Value=0  SampleTime=-1
  Constant1 : Constant  SampleTime=-1
  Sum : Sum  Inputs=|-+
  Switch : Switch  Criteria=u2 > Threshold  SaturateOnIntegerOverflow=off  InputSameDT=off
  Unit Delay : UnitDelay  SampleTime=-1  HasFrameUpgradeWarning=on
  Wait one sample : UnitDelay  SampleTime=-1  HasFrameUpgradeWarning=on
  Out1 : Outport
  wires:
  Unit Delay/1 -> Sum/1
  u/1 -> Unit Delay/1, Sum/2
  1/h2/1 -> Out1/1
  Switch/1 -> 1/h2/1
  Sum/1 -> Switch/1
  Constant/1 -> Switch/3
  Wait one sample/1 -> Switch/2
  Constant1/1 -> Wait one sample/1

== system ssc_hydromech_power_split_cvt_engine_signal_intf/CVT/Other/Port 1 Interface Vehicle/Interface/Discrete/Prediction/Update derivative estimate ==
  u : Inport
  Trigger : TriggerPort  VariantControl=(inherit)
  1/h2 : Gain  Gain=1/h2
  Constant : Constant  Value=0  SampleTime=-1
  Constant1 : Constant  SampleTime=-1
  Sum : Sum  Inputs=|-+
  Switch : Switch  Criteria=u2 > Threshold  SaturateOnIntegerOverflow=off  InputSameDT=off
  Unit Delay : UnitDelay  SampleTime=-1  HasFrameUpgradeWarning=on
  Wait one sample : UnitDelay  SampleTime=-1  HasFrameUpgradeWarning=on
  Out1 : Outport
  wires:
  Unit Delay/1 -> Sum/1
  u/1 -> Unit Delay/1, Sum/2
  1/h2/1 -> Out1/1
  Switch/1 -> 1/h2/1
  Sum/1 -> Switch/1
  Constant/1 -> Switch/3
  Wait one sample/1 -> Switch/2
  Constant1/1 -> Wait one sample/1

== system ssc_hydromech_power_split_cvt_engine_signal_intf/CVT/Simscape/Port 1 Interface Engine/Interface/Discrete/Prediction/Update derivative estimate ==
  u : Inport
  Trigger : TriggerPort  VariantControl=(inherit)
  1/h2 : Gain  Gain=1/h2
  Constant : Constant  Value=0  SampleTime=-1
  Constant1 : Constant  SampleTime=-1
  Sum : Sum  Inputs=|-+
  Switch : Switch  Criteria=u2 > Threshold  SaturateOnIntegerOverflow=off  InputSameDT=off
  Unit Delay : UnitDelay  SampleTime=-1  HasFrameUpgradeWarning=on
  Wait one sample : UnitDelay  SampleTime=-1  HasFrameUpgradeWarning=on
  Out1 : Outport
  wires:
  Constant1/1 -> Wait one sample/1
  Wait one sample/1 -> Switch/2
  Constant/1 -> Switch/3
  Sum/1 -> Switch/1
  Switch/1 -> 1/h2/1
  1/h2/1 -> Out1/1
  u/1 -> Sum/2, Unit Delay/1
  Unit Delay/1 -> Sum/1

== system ssc_hydromech_power_split_cvt_engine_signal_intf/CVT/Simscape/Port 1 Interface Vehicle/Interface/Discrete/Prediction/Update derivative estimate ==
  u : Inport
  Trigger : TriggerPort  VariantControl=(inherit)
  1/h2 : Gain  Gain=1/h2
  Constant : Constant  Value=0  SampleTime=-1
  Constant1 : Constant  SampleTime=-1
  Sum : Sum  Inputs=|-+
  Switch : Switch  Criteria=u2 > Threshold  SaturateOnIntegerOverflow=off  InputSameDT=off
  Unit Delay : UnitDelay  SampleTime=-1  HasFrameUpgradeWarning=on
  Wait one sample : UnitDelay  SampleTime=-1  HasFrameUpgradeWarning=on
  Out1 : Outport
  wires:
  Constant1/1 -> Wait one sample/1
  Wait one sample/1 -> Switch/2
  Constant/1 -> Switch/3
  Sum/1 -> Switch/1
  Switch/1 -> 1/h2/1
  1/h2/1 -> Out1/1
  u/1 -> Sum/2, Unit Delay/1
  Unit Delay/1 -> Sum/1

== stateflow chart ssc_hydromech_power_split_cvt_engine_signal_intf/CVT/Simscape/CVT Ratio Ctrl/Clutch Truth Table ==
  state ClutchLogic
    during:
    [K1Actv,K2Actv,K3Actv,K4Actv,KbActv] = ClutchTable(Range);
    state Rest
      during:
      KvActv = 0;
      KrActv = 0;
    state Fwd
      during:
      KvActv = 1;
      KrActv = 0;
    state Rev
      during:
      KvActv = 0;
      KrActv = 1;
    (default) -> (junction 53)
    (junction 53) -> Rev [order 2] : [CmdVehSpdDir==-1]
    (junction 53) -> Fwd [order 3]
    (junction 53) -> Rest [order 1] : [CmdVehSpdDir==0]
    Fwd -> Rest : [CmdVehSpdDir~=1]
    Rev -> Rest : [CmdVehSpdDir~=-1]
    Rest -> Fwd [order 1] : [CmdVehSpdDir==1]
    Rest -> Rev [order 2] : [CmdVehSpdDir==-1]
  data: R function_input; K1 function_output; K2 function_output; K3 function_output; K4 function_output; Kb function_output; Range input; K1Actv output; K2Actv output; K3Actv output; K4Actv output; KbActv output; KvActv output; KrActv output; CmdVehSpdDir input
  function [K1,K2,K3,K4,Kb] = ClutchTable(R):
    | function [K1,K2,K3,K4,Kb] = ClutchTable(R)
    | 
    | aVarTruthTableCondition_1 = false;
    | aVarTruthTableCondition_2 = false;
    | aVarTruthTableCondition_3 = false;
    | aVarTruthTableCondition_4 = false;
    | 
    | 
    | % Range1
    | 
    | aVarTruthTableCondition_1 = logical(R == 1);
    | 
    | % Range2
    | 
    | aVarTruthTableCondition_2 = logical(R == 2);
    | 
    | % Range3
    | 
    | aVarTruthTableCondition_3 = logical(R == 3);
    | 
    | % Range4
    | 
    | aVarTruthTableCondition_4 = logical(R == 4);
    | 
    | if (aVarTruthTableCondition_1 && ~aVarTruthTableCondition_2 && ~aVarTruthTableCondition_3 && ~aVarTruthTableCondition_4)
    |     A1();
    | elseif (~aVarTruthTableCondition_1 && aVarTruthTableCondition_2 && ~aVarTruthTableCondition_3 && ~aVarTruthTableCondition_4)
    |     A2();
    | elseif (~aVarTruthTableCondition_1 && ~aVarTruthTableCondition_2 && aVarTruthTableCondition_3 && ~aVarTruthTableCondition_4)
    |     A3();
    | elseif (~aVarTruthTableCondition_1 && ~aVarTruthTableCondition_2 && ~aVarTruthTableCondition_3 && aVarTruthTableCondition_4)
    |     A4();
    | else % Default
    |     A5();
    | end
    | 
    | function A1()
    | 
    | % ClutchCtrlR1
    | 
    | K1 = 1; K2 = 0; K3 = 0; K4 = 0; Kb = 1;
    | 
    | function A2()
    | 
    | % ClutchCtrlR2
    | 
    | K1 = 0; K2 = 1; K3 = 0; K4 = 0; Kb = 1;
    | 
    | function A3()
    | 
    | % ClutchCtrlR3
    | 
    | K1 = 0; K2 = 1; K3 = 1; K4 = 0; Kb = 0;
    | 
    | function A4()
    | 
    | % ClutchCtrlR4
    | 
    | K1 = 0; K2 = 1; K3 = 0; K4 = 1; Kb = 0;
    | 
    | function A5()
    | 
    | % Default
    | 
    | K1 = 0; K2 = 0; K3 = 0; K4 = 0; Kb = 0;
